simulink model "DSimulator_R2023a"  (R2023a)
settings: Solver=FixedStepAuto  StartTime=0  StopTime=1000  FixedStep=0.004  RelTol=1e-3  EnableMultiTasking=on
undefined symbols (not defined in the file or in its folder): Dynamic, simpleplot, Tau, TrajGen
libraries: simulink x4
settings Model: Creator=E. Dean  LastModifiedBy=glf
settings SolverCC: AlgebraicLoopSolver=TrustRegion
settings DataIOCC: LimitDataPoints=on  SaveFormat=Array  SignalLoggingSaveFormat=ModelDataLogs  ReturnWorkspaceOutputs=off
settings OptimizationCC: ExpressionDepthLimit=2147483647  LifeSpan=inf
settings DebuggingCC: UnderspecifiedInitializationDetection=Classic  MergeDetectMultiDrivingBlocksExec=none  SolverPrmCheckMsg=warning  FcnCallInpInsideContextMsg=warning  UnconnectedInputMsg=warning  UnconnectedOutputMsg=warning  UnconnectedLineMsg=warning  AllowSymbolicDim=off  StateNameClashWarn=warning  SFUnexpectedBacktrackingDiag=warning  SFNoUnconditionalDefaultTransitionDiag=warning  SFExecutionAtInitializationDiag=none  ArithmeticOperatorsInVariantConditions=warning
settings HardwareCC: ProdBitPerPointer=32  ProdBitPerSizeT=32  ProdBitPerPtrDiffT=32  ProdLargestAtomicFloat=None  ProdIntDivRoundTo=Undefined  ProdEndianess=Unspecified  ProdWordSize=32  ProdHWDeviceType=32-bit Generic
settings ModelReferenceCC: EnableRefExpFcnMdlSchedulingChecks=on  PropagateSignalLabelsOutOfModel=off
settings SFSimCC: SimUseLocalCustomCode=off  CustomCodeUndefinedFunction=UseInterfaceOnly
settings RTWCC: RTWUseLocalCustomCode=off
settings CodeAppCC: StateflowObjectComments=on
settings GRTTargetCC: TargetLangStandard=C89/C90 (ANSI)  CombineOutputUpdateFcns=off  GRTInterface=on
settings ConfigComp: CovMetricSettings=dw  CovSaveCumulativeToWorkspaceVar=on  CovSaveSingleToWorkspaceVar=on  CovExternalEMLEnable=off  CovSFcnEnable=off

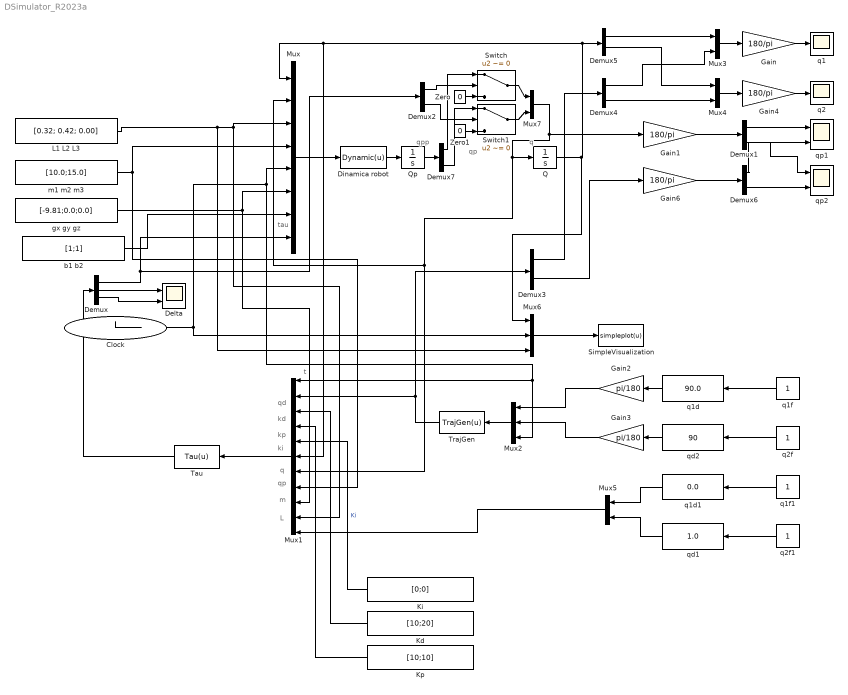
== system DSimulator_R2023a ==
  note: qd
  note: q
  note: qp
  note: qpp
  note: tau
  note: t
  note: L
  note: m
  note: kp
  note: kd
  note: qp
  note: q
  note: ki
  Clock : Clock
  Delta : Scope  NumInputPorts=2
  Demux : Demux  Outputs=3
  Demux{1..7} (7 alike) : Demux  Outputs=2
  Dinamica robot : MATLABFcn  MATLABFcn=Dynamic(u)  OutputDimensions=2
  Gain{,1,4,6} (4 alike) : Gain  Gain=180/pi
  Gain2 : Gain  Gain=pi/180
  Gain3 : Gain  Gain=pi/180
  "Kd " : Constant  Value=[10;20]
  Ki : Constant  Value=[0;0]
  Kp : Constant  Value=[10;10]
  L1 L2 L3 : Constant  Value=[0.32; 0.42; 0.00]
  Mux : Mux  Inputs=8
  Mux1 : Mux  Inputs=11
  Mux2 : Mux  Inputs=3
  Mux{3..5,7} (4 alike) : Mux  Inputs=2
  Mux6 : Mux  Inputs=3
  Q : Integrator  InitialCondition=[0;0]
  Qp : Integrator  InitialCondition=[0;0]
  SimpleVisualization : MATLABFcn  MATLABFcn=simpleplot(u)  OutputDimensions=0
  Switch : Switch  Criteria=u2 ~= 0  SaturateOnIntegerOverflow=off  InputSameDT=off
  Switch1 : Switch  Criteria=u2 ~= 0  SaturateOnIntegerOverflow=off  InputSameDT=off
  "Tau " : MATLABFcn  MATLABFcn=Tau(u)  OutputDimensions=6
  TrajGen : MATLABFcn  MATLABFcn=TrajGen(u)  OutputDimensions=4
  Zero : Constant  Value=0  OutDataTypeStr=Inherit: Inherit via back propagation
  Zero1 : Constant  Value=0  OutDataTypeStr=Inherit: Inherit via back propagation
  b1 b2 : Constant  Value=[1;1]
  gx gy gz : Constant  Value=[-9.81;0.0;0.0]
  "m1 m2 m3 " : Constant  Value=[10.0;15.0]
  q1 : Scope
  q1d : simulink/Math Operations/Slider Gain  gain=90.0  low=-90  high=90
  q1d1 : simulink/Math Operations/Slider Gain  gain=0.0  low=-1  high=1
  q1f : Constant
  q1f1 : Constant
  q2 : Scope
  q2f : Constant
  q2f1 : Constant
  qd1 : simulink/Math Operations/Slider Gain  gain=1.0  low=-1  high=1
  qd2 : simulink/Math Operations/Slider Gain  gain=90  low=-90  high=90
  qp1 : Scope  NumInputPorts=2
  qp2 : Scope  NumInputPorts=2
  wires:
  Dinamica robot/1 -> Qp/1
  Gain/1 -> q1/1
  Gain1/1 -> Demux1/1
  Demux1/1 -> qp1/1
  Demux1/2 -> qp2/1
  Mux/1 -> Dinamica robot/1
  Mux1/1 -> "Tau "/1
  TrajGen/1 -> Demux3/1, Mux1/2
  q1f/1 -> q1d/1
  q2f/1 -> qd2/1
  Mux2/1 -> TrajGen/1
  q1d/1 -> Gain2/1
  Gain3/1 -> Mux2/2
  "Kd "/1 -> Mux1/3
  Kp/1 -> Mux1/4
  Q/1 -> Mux6/1, Mux1/6, Mux/1, Demux5/1
  Qp/1 -> Demux7/1
  "m1 m2 m3 "/1 -> Mux1/8, Mux/4
  L1 L2 L3/1 -> Mux6/3, Mux1/10, Mux/3
  Clock/1 -> Mux2/3, Mux1/1, Mux/5, Mux6/2
  Ki/1 -> Mux1/5  "Ki"
  Demux4/1 -> Mux3/2
  Mux3/1 -> Gain/1
  Gain4/1 -> q2/1
  Mux4/1 -> Gain4/1
  Demux5/1 -> Mux3/1
  Demux5/2 -> Mux4/1
  Demux3/1 -> Demux4/1
  Mux6/1 -> SimpleVisualization/1
  Demux4/2 -> Mux4/2
  Demux3/2 -> Gain6/1
  Demux6/1 -> qp1/2
  Demux6/2 -> qp2/2
  "Tau "/1 -> Demux/1
  Gain2/1 -> Mux2/1
  qd2/1 -> Gain3/1
  Gain6/1 -> Demux6/1
  Demux/1 -> Demux2/1, Mux/8
  gx gy gz/1 -> Mux1/9, Mux/6
  b1 b2/1 -> Mux/7
  q1f1/1 -> q1d1/1
  q2f1/1 -> qd1/1
  q1d1/1 -> Mux5/1
  qd1/1 -> Mux5/2
  Mux5/1 -> Mux1/11
  Demux/2 -> Delta/1
  Demux/3 -> Delta/2
  Demux2/1 -> Switch/2
  Demux2/2 -> Switch1/2
  Demux7/1 -> Switch/1
  Demux7/2 -> Switch1/1
  Zero/1 -> Switch/3
  Zero1/1 -> Switch1/3
  Switch/1 -> Mux7/1
  Switch1/1 -> Mux7/2
  Mux7/1 -> Mux/2, Mux1/7, Q/1, Gain1/1
